simulink model "a24_A_inference_v1"  (R2026a)
settings: Solver=FixedStepDiscrete  StartTime=0  StopTime=23  FixedStep=1
model workspace (MAT data in the model file):
  a24_dictionary = [1  0  0  0  0  0  0  0; 0  1  0  0  0  0  0  0; 0  0  1  0  0  0  0  0; 0  0  0  1  0  0  0  0]
  a24_inputs = timeseries
  a24_inputs.Name = 'unnamed'
  a24_inputs.DataInfo = tsdata.datametadata
  a24_inputs.DataInfo.Interpolation = tsdata.interpolation
  a24_inputs.DataInfo.Interpolation.Fhandle : function handle (value not decoded)
  a24_inputs.DataInfo.Interpolation.Name = 'linear'
  a24_inputs.TimeInfo = tsdata.timemetadata
  a24_inputs.TimeInfo.Length = 24
  a24_inputs.TimeInfo.DuplicateTimes = 0
  a24_inputs.TimeInfo.Time_ = [0; 1; 2; 3; 4; 5; 6; 7; 8; 9; 10; 11; 12; 13; 14; 15; 16; 17; 18; 19; 20; 21; 22; 23]
  a24_inputs.TimeInfo.Initialized = 1
  a24_inputs.QualityInfo = tsdata.qualmetadata
  a24_inputs.Data_ = [3026.659  81.2  1  1  0  0; 2218.177  78.3  1  1  0  0; 2902.304  81  1  1  0  0; 2193.91933333  77.9  1  1  0  0; 2808.14466667  81.3  1  1  0  0; 2120.17766667  75.1  1  1  0  0; 3824.575  80  1  1  0  0; 2700.98066667  75.7  1  1  0  0; 3026.659  81.2  1  0  1  0; 2205.66033333  74.9  1  0  1  0; 2902.304  81  1  0  1  0; 2112.29733333  72.9  1  0  1  0; 2808.14466667  81.3  1  0  1  0; 2092.628  71.7  1  0  1  0; 3824.575  80  1  0  1  0; 2542.90933333  73.8  1  0  1  0; 3026.659  81.2  1  0  0  1; 3382.50466667  75  1  0  0  1; 2902.304  81  1  0  0  1; 2413.05233333  73.3  1  0  0  1; 2808.14466667  81.3  1  0  0  1; 2538.15333333  73  1  0  0  1; 3824.575  80  1  0  0  1; 3938.38166667  73.7  1  0  0  1]
  a24_kind = 1
  a24_mean = [2625.56568519 77.2222222222]
  a24_scale = [585.088406321 4.03273116323]
  a24_weights = [-4.04071511288; 0.689988453793; 0.812982593616; -2.58577674472; -0.438344206427; 0.267005033857; 2.5069612389; 5.51846500849; -0.156507155123; -1.82324338075; -2.56687041337; -3.55560781971; 4.8872956794; -2.18935510504; -0.963817873277; 4.95194802973; -0.580075864141; 1.02232671479; 2.60376628403; 0.850219955467; -1.54455634376; 1.24559065941; 3.71560276241; 1.0518662402; -3.72753301852; 1.6492821301; 1.39805798654; -3.90031066119; 0.293920277924; 0.317010276704; 3.08991247033; 0.399804125195; 0.0955895441478; 0.324783943118; 3.19679129309; 0.370447743519; 0.28818959172; 0.343325388861; 3.09303361383; 0.429092128737; -0.00225658022848; 0.318724778273; 3.2292225395; 0.347905711966; 2.38324843017; -4.27324205517; -3.13315379789; -1.28935444452; -3.02613685725; -3.00571771941; -2.97255641045; -3.04000768828]
Description:
  | Frozen A24 TaskIL onehot/no-negotiation/seed101/stage3 example;24 reporting views of16 average records. Tick=record order, not physical time. Full55-checkpoint1040-view parity is separate. No online training, new physical validation or blind test.
settings Model: Creator=salih  LastModifiedBy=salih

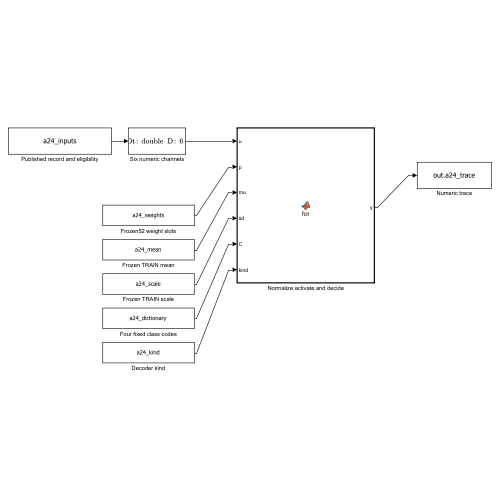
[thumbnail: Simulink's stored preview of the top-level diagram]
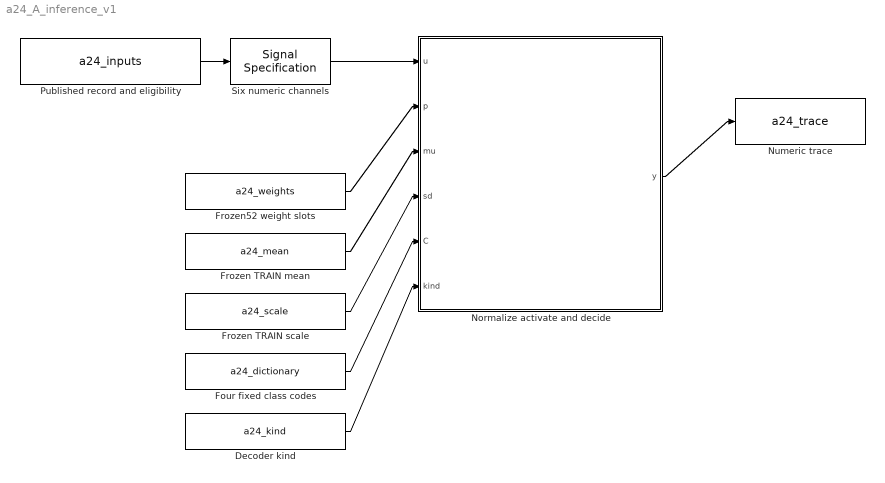
== system a24_A_inference_v1 ==
  Decoder kind : Constant  Value=a24_kind
  Four fixed class codes : Constant  Value=a24_dictionary
  Frozen TRAIN mean : Constant  Value=a24_mean
  Frozen TRAIN scale : Constant  Value=a24_scale
  Frozen52 weight slots : Constant  Value=a24_weights
  Normalize activate and decide : MATLAB Function  TreatAsAtomicUnit=on
  Numeric trace : ToWorkspace  VariableName=a24_trace  SampleTime=1
  Published record and eligibility : FromWorkspace  VariableName=a24_inputs  SampleTime=1  Interpolate=off  OutputAfterFinalValue=Holding final value
  Six numeric channels : SignalSpecification  OutDataTypeStr=double  Dimensions=6
  wires:
  Published record and eligibility/1 -> Six numeric channels/1
  Six numeric channels/1 -> Normalize activate and decide/1(u)
  Frozen52 weight slots/1 -> Normalize activate and decide/2(p)
  Frozen TRAIN mean/1 -> Normalize activate and decide/3(mu)
  Frozen TRAIN scale/1 -> Normalize activate and decide/4(sd)
  Four fixed class codes/1 -> Normalize activate and decide/5(C)
  Decoder kind/1 -> Normalize activate and decide/6(kind)
  Normalize activate and decide/1(y) -> Numeric trace/1

== matlab function a24_A_inference_v1/Normalize activate and decide ==
  data: u input; y output; p input; mu input; sd input; C input; kind input
function y = fcn(u,p,mu,sd,C,kind)
%#codegen
% Frozen A24 recognition. u=[E,ShoreD,eligible1..4]; kind1=code,2=CE.
% Fixed52 weight slots, codebook4x8. No truth/row/model identity input.
% y18=[normalized2,activation8,active_scores4,gap,forced,tie,status].
% Scores: code=-mean squared distance; CE=eligible softmax.
% CE unused activation slots and inactive class scores are NaN.
y=nan(1,18);y(16)=0;y(17)=0;y(18)=-1;
u=reshape(u,1,6);p=reshape(p,52,1);mu=reshape(mu,1,2);sd=reshape(sd,1,2);
if any(~isfinite([u,p',mu,sd])) || any(sd<=0) || ~(kind==1 || kind==2)
 return;
end
mask=u(3:6);
if any(~(mask==0 | mask==1)) || sum(mask)<2,return;end
if kind==1 && (any(~isfinite(C(:))) || any(~(C(:)==0 | C(:)==1)))
 return;
end
x=(u(1:2)-mu)./sd;
h=tanh(x*reshape(p(1:8),2,4)+reshape(p(9:12),1,4));
activation=nan(1,8);score=-inf(1,4);
if kind==1
 logits8=h*reshape(p(13:44),4,8)+reshape(p(45:52),1,8);
 if any(~isfinite(logits8)),return;end
 for b=1:8
  if logits8(b)>=0
   activation(b)=1/(1+exp(-logits8(b)));
  else
   eb=exp(logits8(b));activation(b)=eb/(1+eb);
  end
 end
 for k=1:4
  if mask(k)==1,score(k)=-sum((activation-C(k,:)).^2)/8;end
 end
else
 % CE uses its original contiguous32 slots; slots33..52 are unused zeros.
 logits4=h*reshape(p(13:28),4,4)+reshape(p(29:32),1,4);
 if any(~isfinite(logits4)),return;end
 top=-inf;
 for k=1:4,if mask(k)==1 && logits4(k)>top,top=logits4(k);end,end
 ex=zeros(1,4);
 for k=1:4,if mask(k)==1,ex(k)=exp(logits4(k)-top);end,end
 probability=ex/sum(ex);activation(1:4)=probability;
 for k=1:4,if mask(k)==1,score(k)=probability(k);end,end
end
best=-inf;second=-inf;forced=0;
for k=1:4
 if mask(k)==1
  if score(k)>best
   second=best;best=score(k);forced=k;
  elseif score(k)>second
   second=score(k);
  end
 end
end
tieCount=0;
for k=1:4,if mask(k)==1 && score(k)==best,tieCount=tieCount+1;end,end
if ~isfinite(best) || ~isfinite(second) || any(~isfinite(x)),return;end
y(1:2)=x;y(3:10)=activation;
for k=1:4,if mask(k)==1,y(10+k)=score(k);end,end
y(15)=best-second;y(16)=forced;y(17)=double(tieCount>1);y(18)=1;
end
